simulink model "NBMS_SoC"  (R2026b)
settings: Solver=FixedStepDiscrete  StopTime=25  FixedStep=0.1
undefined symbols (not defined in the file): BMS_BattSoCDerate_E, BMS_BattTempDerate_E, BMS_MODE_E, CAL_15_SOC_WRN_RVL_THRSH, CAL_15_SOC_WRN_THRSH, CAL_DCHRG_END_THRSH, CAL_DOD, CAL_DOD_MAX_THRSH, CAL_DOD_MIN_THRSH, CAL_ENABLE_SOC_WARN_15, CAL_ENABLE_SOC_WARN_20, CAL_GOLDEN_CHARGE, CAL_GOLDEN_DC, CAL_LOW_SOC_RVL_THRSH, CAL_LOW_SOC_THRSH, CAL_NOMINAL_VOLTAGE, CAL_SOC_WRN_RVL_THRSH, CAL_SOC_WRN_THRSH, CAL_SOH_Enable, Charger_Mode_Req_E, DiscIntNeverNeededParam, OBC_E, VDU_MACHINE_STS_E, X_DCIR_CHG, X_DCIR_DISCH, Y_DCIR_CHG, Y_DCIR_DISCH
libraries: simulink x110, simulink_extras x6, sl_discontinuities x3
(part 2 of 3)

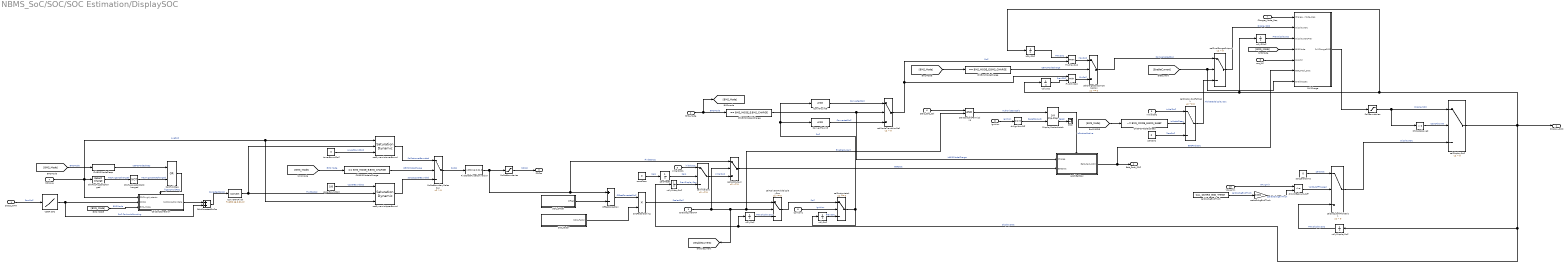
== system NBMS_SoC/SOC/SOC Estimation/DisplaySOC ==
  SOCcc_RAW : Inport
  BMS_Mode : Inport  Port=2
  EnableCurrentMA : Inport  Port=3
  SOCAvg : Inport  Port=4
  InitialSOC : Inport  Port=5
  Start_SOC_Cal : Inport  Port=6
  Charger_Mode_Req : Inport  Port=7
  Ignition : Inport  Port=8
  soc_full : Inport  Port=9
  VtAvgMin : Inport  Port=10
  CalcCorrectedSoCcc : Sum
  CalcSoCCorrection : Subsystem
  ChkBMSMODEIsSleep : simulink/Logic and Bit Operations/Compare To Constant  relop=~=  const=BMS_MODE_E.BMS_SLEEP  OutDataTypeStr=boolean
  ChkBMSModeIsCharge : simulink/Logic and Bit Operations/Compare To Constant  relop===  const=BMS_MODE_E.BMS_CHARGE  OutDataTypeStr=boolean
  ChkBMSModeSleep : simulink/Logic and Bit Operations/Compare To Constant  relop===  const=BMS_MODE_E.BMS_SLEEP  OutDataTypeStr=boolean
  ChkBMSModeisCharge : simulink/Logic and Bit Operations/Compare To Constant  relop===  const=BMS_MODE_E.BMS_CHARGE  OutDataTypeStr=boolean
  ChkBmsModeCharge : simulink/Logic and Bit Operations/Compare To Constant  relop===  const=BMS_MODE_E.BMS_CHARGE  OutDataTypeStr=boolean
  ChkHasAvgSoCChanged : simulink/Logic and Bit Operations/Detect Change  vinit=0  OutDataTypeStr=boolean
  ChkHasAvgSoCNotChanged : Logic  Operator=NOT  AllPortsSameDT=off  OutDataTypeStr=boolean
  ChkSoCabove0 : simulink/Logic and Bit Operations/Compare To Constant  relop=>  const=0  OutDataTypeStr=boolean
  ConvertToFixdt : DataTypeConversion  OutDataTypeStr=fixdt(0,16,0.01,0)  RndMeth=Floor
  ConvertTouin8 : DataTypeConversion  OutDataTypeStr=uint8  RndMeth=Ceiling
  ConvtTouint8 : DataTypeConversion  OutDataTypeStr=uint8  RndMeth=Floor
  DisplaySocLockLatch : simulink_extras/Flip Flops/S-R Flip-Flop  initial_condition=0
  FindMaxSoC : MinMax  Function=max  Inputs=2
  FindMinSoC : MinMax  Inputs=2
  FixdtDataTypeConversion : DataTypeConversion  OutDataTypeStr=fixdt(0,16,0.01,0)  RndMeth=Floor
  FullCharge : Subsystem
  GND : Terminator
  Ignition1 : InportShadow  Port=8
  InitialSOC1 : InportShadow  Port=5
  LatchBattSoc : Subsystem
  LowerBoundSoC : Constant  Value=0  OutDataTypeStr=fixdt(0,16,0.01,0)
  OffsetCorrection : Sum  Inputs=+-
  SOC_Offset : Subsystem
  SOC_factor : Subsystem
  SoCBoundaries : Saturate  UpperLimit=100  LowerLimit=0  OutDataTypeStr=uint8  RndMeth=Ceiling
  SoCFactorScaling : Product
  SoCHoldReq : Logic  Operator=OR  AllPortsSameDT=off  OutDataTypeStr=boolean
  SoCZeroClamp : Constant  Value=0  OutDataTypeStr=uint8
  SoCccBoundaries : Saturate  UpperLimit=100  LowerLimit=0  RndMeth=Nearest
  SoCccBoundarySelection : Switch  Criteria=u2 > Threshold  SaturateOnIntegerOverflow=off  InputSameDT=off
  StartSocCalcPermissive : Logic  AllPortsSameDT=off  OutDataTypeStr=boolean
  UDlySOC : UnitDelay  SampleTime=-1
  USER SOC : Lookup_n-D  NumberOfTableDimensions=1  BreakpointsForDimension1=[0,100]  Table=[0,100]  InternalRulePriority=Speed  RndMeth=Simplest
  UdlySoc : UnitDelay  SampleTime=-1
  UpperBoundSoC : Constant  Value=100  OutDataTypeStr=fixdt(0,16,0.01,0)
  ZeroReset : UnitDelay  InitialCondition=1  SampleTime=-1
  ZeroSoC : Constant  Value=0  OutDataTypeStr=uint8
  calDischgEndThrsh : Constant  Value=CAL_DCHRG_END_THRSH
  chkIgnitionOff : simulink/Logic and Bit Operations/Compare To Constant  relop===  const=0  OutDataTypeStr=boolean
  chkVoltBelowCutoff : RelationalOperator  Operator=<=  OutDataTypeStr=boolean  RndMeth=Simplest  InputSameDT=off
  constZero : Constant  Value=0  OutDataTypeStr=boolean
  satDynamicLowerBound : sl_discontinuities/Saturation Dynamic  OutMin=[]  OutMax=[]  OutDataTypeStr=Inherit: Same as second input  OutDataType=fixdt(1, 16)  OutScaling=2^-10  DoSatur=off
  satDynamicUpperBound : sl_discontinuities/Saturation Dynamic  OutMin=[]  OutMax=[]  OutDataTypeStr=Inherit: Same as second input  OutDataType=fixdt(1, 16)  OutScaling=2^-10  DoSatur=off
  scaleDchgEndThrsh : Gain  Gain=0.001
  selActiveOrHoldDisplaySoc : Switch  Criteria=u2 ~= 0  SaturateOnIntegerOverflow=off  InputSameDT=off
  selChargeSocCompensation : Switch  Criteria=u2 ~= 0  SaturateOnIntegerOverflow=off  InputSameDT=off
  selDisplaySoC : Switch  Criteria=u2 > Threshold  SaturateOnIntegerOverflow=off  InputSameDT=off
  selDisplaySocFallback : Switch  Criteria=u2 ~= 0  SaturateOnIntegerOverflow=off  InputSameDT=off
  selFinalGaugeOutput : Switch  Criteria=u2 > Threshold  SaturateOnIntegerOverflow=off  InputSameDT=off
  selInitialSoc : Switch  Criteria=u2 ~= 0  SaturateOnIntegerOverflow=off  InputSameDT=off
  selModeTransitionRef : Switch  Criteria=u2 > Threshold  SaturateOnIntegerOverflow=off  InputSameDT=off
  selSoCOutput : Switch  Criteria=u2 ~= 0  SaturateOnIntegerOverflow=off  InputSameDT=off
  selSocCutoffArbitration : Switch  Criteria=u2 > Threshold  SaturateOnIntegerOverflow=off  InputSameDT=off
  selSocIgnLatch : Switch  Criteria=u2 ~= 0  SaturateOnIntegerOverflow=off  InputSameDT=off
  uDlySoC : UnitDelay  InitialCondition=100  SampleTime=-1
  udlyDSoC : UnitDelay  InitialCondition=100  SampleTime=-1
  udlyDislaySoC : UnitDelay  SampleTime=-1
  udlyDisplaySoC : UnitDelay  SampleTime=-1
  udlySoC : UnitDelay  SampleTime=-1
  Display_SOC : Outport
  Batt_Pack_SOC : Outport  Port=2
  SOCcc : Outport  Port=3
  wires:
  [BMS_Mode] -> ChkBMSModeSleep/1  "BMSMode"
  ChkBMSModeSleep/1 -> SoCHoldReq/1  "IsBMSModeSleep"
  SoCHoldReq/1 -> CalcSoCCorrection/Enable  "flgSoCHoldReq"
  ChkHasAvgSoCNotChanged/1 -> SoCHoldReq/2  "HasAvgSoCNotChanged"
  [BMS_Mode] -> CalcSoCCorrection/3(BMS_Mode)  "BMSMode"
  soc_full/1 -> FullCharge/5(soc_full)
  udlySoC/1 -> selSocIgnLatch/3  "PrevSoC"
  selActiveOrHoldDisplaySoc/1 -> selSocIgnLatch/1  "SoC"
  Ignition1/1 -> selSocIgnLatch/2  "Ignition"
  [BMS_Mode] -> FullCharge/4(BMSMode)
  selDisplaySocFallback/1 -> selFinalGaugeOutput/3  "ArbitratedDisplaySoc"
  ZeroSoC/1 -> selDisplaySocFallback/3  "ZeroSoC"
  InitialSOC/1 -> selDisplaySocFallback/1  "initialSoC"
  ChkBMSMODEIsSleep/1 -> selDisplaySocFallback/2  "IsModeSleep"
  [BMS_Mode] -> ChkBMSMODEIsSleep/1
  uDlySoC/1 -> selActiveOrHoldDisplaySoc/3  "PrevDisplaySoc"
  BMS_Mode/1 -> ChkBMSModeisCharge/1, [BMS_Mode]  "BMSMode"
  LatchBattSoc/1(Batt_Pack_SOC) -> FullCharge/6(Batt_Pack_SOC), Batt_Pack_SOC/1  "BattPackSoC"
  Ignition/1 -> chkIgnitionOff/1  "Ignition"
  chkIgnitionOff/1 -> DisplaySocLockLatch/2  "ResetSocLock"
  udlyDSoC/1 -> FullCharge/3(DisplaySOCPrev)  "PrevDisplaySoc"
  Charger_Mode_Req/1 -> FullCharge/1(Charger_Mode_Req)
  FullCharge/1(FullChargeSOC) -> SoCBoundaries/1
  ConvertToFixdt/1 -> satDynamicLowerBound/2, satDynamicUpperBound/2  "FixdtSoCcc"
  UpperBoundSoC/1 -> satDynamicUpperBound/1  "UpperBoundSoc"
  satDynamicUpperBound/1 -> SoCccBoundarySelection/3  "SoCccUpperBounded"
  LowerBoundSoC/1 -> satDynamicLowerBound/3  "LowerBoundSoC"
  CalcCorrectedSoCcc/1 -> ConvertToFixdt/1  "CorrectedSoCcc"
  satDynamicLowerBound/1 -> SoCccBoundarySelection/1  "SoCccLowerBounded"
  ChkBMSModeIsCharge/1 -> SoCccBoundarySelection/2  "IsBMSModeCharge"
  [BMS_Mode] -> ChkBMSModeIsCharge/1  "BMS Mode"
  StartSocCalcPermissive/1 -> DisplaySocLockLatch/1  "AuthorizeSocCalc"
  Start_SOC_Cal/1 -> StartSocCalcPermissive/1
  DisplaySocLockLatch/2 -> GND/1  "Reset"
  DisplaySocLockLatch/1 -> LatchBattSoc/Enable  "IsSocLockActive"
  selSoCOutput/1 -> LatchBattSoc/2(BattSOC)  "BattSoC"
  constZero/1 -> ZeroReset/1  "Zero"
  ZeroReset/1 -> selInitialSoc/2  "Zero"
  InitialSOC1/1 -> selInitialSoc/1  "initialSoC"
  selInitialSoc/1 -> selSoCOutput/3  "InitialSoC"
  ChkBMSModeisCharge/1 -> LatchBattSoc/1(Charge), selModeTransitionRef/2  "IsBMSModeCharge"
  SoCccBoundaries/1 -> SOCcc/1  "SOCcc"
  [EnableCurrent] -> selFinalGaugeOutput/2, FullCharge/7(Enable2sec)
  USER SOC/1 -> CalcCorrectedSoCcc/2, CalcSoCCorrection/2(SOCcc)  "SoC CoulombCounting"
  selFinalGaugeOutput/1 -> FullCharge/2(DisplaySOC)  "DisplaySOC"
  selChargeSocCompensation/1 -> selFinalGaugeOutput/1  "CompensatedSoc"
  UdlySoc/1 -> FindMinSoC/2  "PrevSOC"
  UDlySOC/1 -> FindMaxSoC/1  "PrevSoC"
  selModeTransitionRef/1 -> FindMaxSoC/2, FindMinSoC/1  "SoC"
  FindMinSoC/1 -> selChargeSocCompensation/3  "MinSoC"
  FindMaxSoC/1 -> selChargeSocCompensation/1  "MaxSoC"
  [BMS_Mode] -> ChkBmsModeCharge/1
  ChkBmsModeCharge/1 -> selChargeSocCompensation/2  "IsBmsModeCharge"
  CalcSoCCorrection/1(SoCCorrectionRate) -> CalcCorrectedSoCcc/1
  ChkHasAvgSoCChanged/1 -> ChkHasAvgSoCNotChanged/1  "HasAvgSoCChanged"
  udlyDislaySoC/1 -> selInitialSoc/3  "PrevDisplaySoc"
  FixdtDataTypeConversion/1 -> OffsetCorrection/1, selSoCOutput/1, SoCccBoundaries/1  "FixdtSoCcc"
  ConvertTouin8/1 -> selModeTransitionRef/3  "ConvertedSoC"
  ConvtTouint8/1 -> selModeTransitionRef/1  "ConvertedSoC"
  selSocIgnLatch/1 -> ConvertTouin8/1, ConvtTouint8/1, udlySoC/1  "SoC"
  SoCFactorScaling/1 -> selActiveOrHoldDisplaySoc/1  "ScaledSoC"
  EnableCurrentMA/1 -> selSoCOutput/2, selActiveOrHoldDisplaySoc/2, StartSocCalcPermissive/2, [EnableCurrent]  "EnableCurrent"
  udlyDisplaySoC/1 -> selSocCutoffArbitration/3  "PrevDisplaySoC"
  SoCZeroClamp/1 -> selSocCutoffArbitration/1  "ZeroSoC"
  selSocCutoffArbitration/1 -> selDisplaySoC/3  "DisplaySOC"
  ChkSoCabove0/1 -> selDisplaySoC/2  "IsSoCAbove0"
  SoCBoundaries/1 -> ChkSoCabove0/1, selDisplaySoC/1  "DisplaySOC"
  SOCcc_RAW/1 -> USER SOC/1  "RawSoC"
  SOCAvg/1 -> ChkHasAvgSoCChanged/1, satDynamicLowerBound/1, satDynamicUpperBound/3, CalcSoCCorrection/1(SOCAvgHystersis)  "AvgSoC"
  selDisplaySoC/1 -> udlyDislaySoC/1, uDlySoC/1, udlyDisplaySoC/1, UDlySOC/1, udlyDSoC/1, UdlySoc/1, Display_SOC/1  "DisplaySOC"
  SOC_factor/1(SOC_Factor) -> SoCFactorScaling/2
  SOC_Offset/1(Offset) -> OffsetCorrection/2
  OffsetCorrection/1 -> SoCFactorScaling/1  "OffsetCorrectedSoC"
  SoCccBoundarySelection/1 -> FixdtDataTypeConversion/1  "SoCcc"
  calDischgEndThrsh/1 -> scaleDchgEndThrsh/1  "calDischgEndThrsh"
  scaleDchgEndThrsh/1 -> chkVoltBelowCutoff/2  "scaledDchgenThrsh"
  chkVoltBelowCutoff/1 -> selSocCutoffArbitration/2  "VoltCutoffTripped"
  VtAvgMin/1 -> chkVoltBelowCutoff/1  "VtAvgmin"

== system NBMS_SoC/SOC/SOC Estimation/LatchTempinit ==
  Temp : Inport
  Ignition : TriggerPort  VariantControl=(inherit)
  Temp_Init : Outport
  wires:
  Temp/1 -> Temp_Init/1

== system NBMS_SoC/SOC/SOC Estimation/SOC Overriding Handling ==
  soc_full : Inport
  Real_SOC : Inport  Port=2
  DisCharging_SOC : Inport  Port=3
  Charger_Mode_Req : Inport  Port=4
  BMS_Mode : Inport  Port=5
  CalcChgSoC : Sum  Inputs=+-
  ChkBMSModeSleep : simulink/Logic and Bit Operations/Compare To Constant  relop===  const=BMS_MODE_E.BMS_SLEEP  OutDataTypeStr=boolean
  ChkChgModeReqChgComplete : simulink/Logic and Bit Operations/Compare To Constant  relop===  const=Charger_Mode_Req_E.Charge_Complete  OutDataTypeStr=boolean
  ChkChgModeReqDisabled : simulink/Logic and Bit Operations/Compare To Constant  relop===  const=Charger_Mode_Req_E.Disabled  OutDataTypeStr=boolean
  LatchSoC : Subsystem  TreatAsAtomicUnit=on
  SoCccBoundaries : Saturate  UpperLimit=100  LowerLimit=0  OutDataTypeStr=double  RndMeth=Nearest
  SocStateController : Stateflow chart  TreatAsAtomicUnit=on
      settings: PortSchema="{\"entries\":[{\"content\":{\"sides\":[{\"content\":{\"connectorIds\":[\"In2\",\"In3\",\"In1\"]},\"type\":\"ConnectorPlacement.EquallySpacedRectSide\",\"uuid\":\"4d9dda48-5fd1-41f9-94f0-c80678ed5835\"},{\"content\":{\"connectorIds\":[\"Out1\"],\"side\":\"RIGHT\"},\"type\":\"ConnectorPlacement.EquallySpacedRectSide\",\"uuid\":\"c790fe46-1928-4eaf-b04a-be0eaec66a70\"},{\"content\":{\"side\":\"TOP\"},\"type\":\"ConnectorPlacement.EquallySpacedRectSide\",\"uuid\":\"e10142f7-42dd-412d-a45a-7f68ca23bebc\"},{\"content\":{\"side\":\"BOTTOM\"},\"type\":\"ConnectorPlacement.EquallySpacedRectSide\",\"uuid\":\"e986da1d-d2bc-437c-8de3-8b77989038a9\"}]},\"type\":\"ConnectorPlacement.EquallySpacedConnector\",\"uuid\":\"0a51b432-3f9b-4bde-863c-799f895a3b2c\"}],\"packageUris\":[\"http://schema.mathworks.com/mf0/Connector/R2020b\"],\"version\":\"1.0\"}"
  selChgOrRealSoc : Switch  Criteria=u2 > Threshold  SaturateOnIntegerOverflow=off  InputSameDT=off
  SOC_CC : Outport
  wires:
  CalcChgSoC/1 -> selChgOrRealSoc/1  "ChgSoC"
  LatchSoC/1(SOC) -> CalcChgSoC/1
  soc_full/1 -> LatchSoC/1(SOC_Full)  "SoCfull"
  ChkBMSModeSleep/1 -> SocStateController/3(BMS_sleep)  "IsBmsModeSleep"
  BMS_Mode/1 -> ChkBMSModeSleep/1
  SoCccBoundaries/1 -> SOC_CC/1  "SoCcc"
  selChgOrRealSoc/1 -> SoCccBoundaries/1  "UncappedSoCcc"
  Charger_Mode_Req/1 -> ChkChgModeReqChgComplete/1, ChkChgModeReqDisabled/1  "ChgModeReq"
  ChkChgModeReqDisabled/1 -> SocStateController/2(D)  "IsChgModeReqDisabled"
  SocStateController/1(A) -> selChgOrRealSoc/2  "SocSourceControl"
  Real_SOC/1 -> selChgOrRealSoc/3  "SoC"
  DisCharging_SOC/1 -> CalcChgSoC/2  "DischgSoc"
  ChkChgModeReqChgComplete/1 -> SocStateController/1(C), LatchSoC/Trigger  "IsChgModeReqChgComplete"

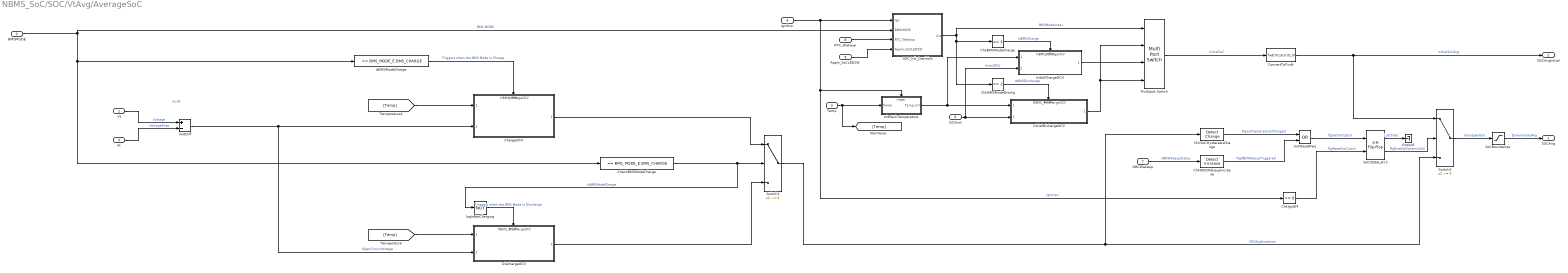
== system NBMS_SoC/SOC/VtAvg/AverageSoC ==
  note: Vt-IR
  Vt : Inport
  BMSMODE : Inport  Port=2
  Temp : Inport  Port=3  OutDataTypeStr=double
  Ignition : Inport  Port=4
  IR : Inport  Port=5
  OCVInit : Inport  Port=6
  OBCWakeup : Inport  Port=7
  RTC_Wakeup : Inport  Port=8
  AppIn_SoCLEDSW : Inport  Port=9
  ChargeOCV : ModelReference  ModelNameDialog=NBMS_ChargeOCV.slx  SimulationMode=Normal  ModelReferenceVersion=7.15  EnablePortName=EnableWhenValid  EnablePortStatesWhenEnabling=reset
  CheckBMSModeCharge : simulink/Logic and Bit Operations/Compare To Constant  relop===  const=BMS_MODE_E.BMS_CHARGE  OutDataTypeStr=boolean
  ChkBMSModeCharge : simulink/Logic and Bit Operations/Compare To Constant  relop===  const=1  OutDataTypeStr=boolean
  ChkBMSModeDischg : simulink/Logic and Bit Operations/Compare To Constant  relop===  const=2  OutDataTypeStr=boolean
  ChkIgnOff : simulink/Logic and Bit Operations/Compare To Zero  relop===  OutDataTypeStr=boolean
  ChkOBCWakeupIncrease : simulink/Logic and Bit Operations/Detect Increase  vinit=0.0  OutDataTypeStr=boolean
  ChkSoCHysteresisChange : simulink/Logic and Bit Operations/Detect Change  vinit=0  OutDataTypeStr=boolean
  ConvertToFixdt : DataTypeConversion  OutDataTypeStr=fixdt(0,16,0.01,0)  SaturateOnIntegerOverflow=off  RndMeth=Floor
  DischargeOCV : ModelReference  ModelNameDialog=NBMS_DischargeOCV.slx  SimulationMode=Normal  ModelReferenceVersion=7.7  EnablePortName=EnableWhenValid  EnablePortStatesWhenEnabling=reset
  Ground : Terminator
  InitPackTemperature : Subsystem  TreatAsAtomicUnit=on
  InitialChargeOCV : ModelReference  ModelNameDialog=NBMS_ChargeOCV.slx  SimulationMode=Normal  ModelReferenceVersion=7.15  EnablePortName=EnableWhenValid  EnablePortStatesWhenEnabling=reset
  InitialDichargeOCV : ModelReference  ModelNameDialog=NBMS_DischargeOCV.slx  SimulationMode=Normal  ModelReferenceVersion=7.7  EnablePortName=EnableWhenValid  EnablePortStatesWhenEnabling=reset
  IsBMSModeCharge : simulink/Logic and Bit Operations/Compare To Constant  relop===  const=BMS_MODE_E.BMS_CHARGE  OutDataTypeStr=boolean
  Multiport Switch : MultiPortSwitch  DataPortOrder=Zero-based contiguous  DiagnosticForDefault=None  zeroidx=on  SaturateOnIntegerOverflow=off  InputSameDT=off
  SOC_Init_Decision : Stateflow chart  TreatAsAtomicUnit=on
  SoCBoundaries : Saturate  UpperLimit=100  LowerLimit=0  RndMeth=Nearest
  SoCResetReq : Logic  Operator=OR  AllPortsSameDT=off  OutDataTypeStr=boolean
  SoCStateLatch : simulink_extras/Flip Flops/S-R Flip-Flop  initial_condition=0
  Switch1 : Switch  Criteria=u2 ~= 0  OutDataTypeStr=fixdt(0,16,0.01,0)  SaturateOnIntegerOverflow=off  InputSameDT=off
  Switch2 : Switch  Criteria=u2 ~= 0  SaturateOnIntegerOverflow=off  InputSameDT=off
  VoltDiff : Sum  Inputs=+-  OutDataTypeStr=fixdt(1,16,0.001,0)  AccumDataTypeStr=fixdt(1,16,0.001,0)
  logIsNotCharging : Logic  Operator=NOT  AllPortsSameDT=off  OutDataTypeStr=boolean
  SOCAvg : Outport
  SOCAvgInitial : Outport  Port=2
  wires:
  Vt/1 -> VoltDiff/1  "Voltage"
  OCVInit/1 -> InitialDichargeOCV/2, InitialChargeOCV/2  "InitialOCV"
  ChkIgnOff/1 -> SoCStateLatch/2  "flgResetSoCLatch"
  ChkBMSModeCharge/1 -> InitialChargeOCV/Enable  "IsBMSCharge"
  ChkOBCWakeupIncrease/1 -> SoCResetReq/2  "FlgOBCWakeupTriggered"
  SoCBoundaries/1 -> SOCAvg/1  "DynamicSoCAvg"
  ChkBMSModeDischg/1 -> InitialDichargeOCV/Enable  "IsBMSDischarge"
  SoCStateLatch/2 -> Switch2/2  "FlgEnableDynamicSoC"
  SoCStateLatch/1 -> Ground/1  "LatchSet"
  BMSMODE/1 -> CheckBMSModeCharge/1, IsBMSModeCharge/1, SOC_Init_Decision/2(BMSMODE)  "BMS MODE"
  Switch1/1 -> Switch2/3, ChkSoCHysteresisChange/1  "SOCAvgHystersis"
  Multiport Switch/1 -> ConvertToFixdt/1  "InitialSoC"
  SOC_Init_Decision/1(Init) -> Multiport Switch/1, ChkBMSModeCharge/1, ChkBMSModeDischg/1  "BMSModeIndex"
  ChkSoCHysteresisChange/1 -> SoCResetReq/1  "FlgSoCHysteresisIsChanged"
  ConvertToFixdt/1 -> Switch2/1, SOCAvgInitial/1  "InitialSoCAvg"
  [Temp] -> ChargeOCV/1
  VoltDiff/1 -> ChargeOCV/2, DischargeOCV/2  "OpenCircuitVoltage"
  Switch2/1 -> SoCBoundaries/1  "UncappedSoc"
  OBCWakeup/1 -> ChkOBCWakeupIncrease/1  "OBCWakeupStatus"
  IR/1 -> VoltDiff/2  "VoltageDrop"
  Ignition/1 -> InitPackTemperature/Trigger, ChkIgnOff/1, SOC_Init_Decision/1(Ign)  "Ignition"
  CheckBMSModeCharge/1 -> logIsNotCharging/1, Switch1/2  "IsBMSModeCharge"
  [Temp] -> DischargeOCV/1
  logIsNotCharging/1 -> DischargeOCV/Enable  "Triggers when the BMS Mode is Discharge"
  IsBMSModeCharge/1 -> ChargeOCV/Enable  "Triggers when the BMS Mode is Charge"
  Temp/1 -> InitPackTemperature/1(Temp), [Temp]
  SoCResetReq/1 -> SoCStateLatch/1  "flgSetSoCLatch"
  InitPackTemperature/1(Temp_Init) -> InitialDichargeOCV/1, InitialChargeOCV/1
  ChargeOCV/1 -> Switch1/1
  DischargeOCV/1 -> Switch1/3
  InitialChargeOCV/1 -> Multiport Switch/3
  InitialDichargeOCV/1 -> Multiport Switch/2, Multiport Switch/4
  RTC_Wakeup/1 -> SOC_Init_Decision/3(RTC_Wakeup)
  AppIn_SoCLEDSW/1 -> SOC_Init_Decision/4(AppIn_SoCLEDSW)

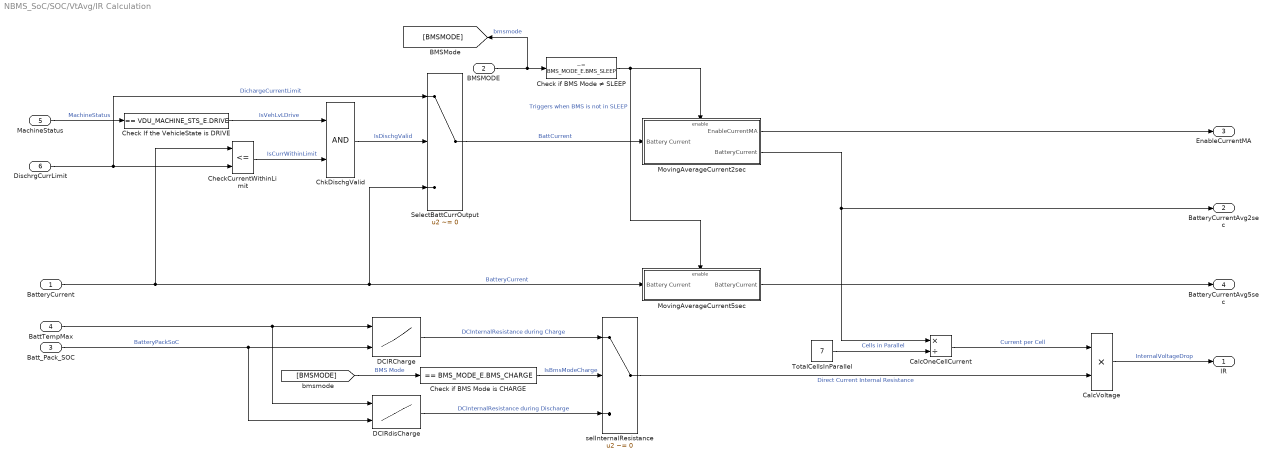
== system NBMS_SoC/SOC/VtAvg/IR Calculation ==
  BatteryCurrent : Inport
  BMSMODE : Inport  Port=2
  Batt_Pack_SOC : Inport  Port=3
  BattTempMax : Inport  Port=4
  MachineStatus : Inport  Port=5  OutDataTypeStr=Enum: VDU_MACHINE_STS_E
  DischrgCurrLimit : Inport  Port=6
  CalcOneCellCurrent : Product  Inputs=*/
  CalcVoltage : Product
  Check If the VehicleState is DRIVE : simulink/Logic and Bit Operations/Compare To Constant  relop===  const=VDU_MACHINE_STS_E.DRIVE  OutDataTypeStr=boolean
  "Check if BMS Mode ≠ SLEEP " : simulink/Logic and Bit Operations/Compare To Constant  relop=~=  const=BMS_MODE_E.BMS_SLEEP  OutDataTypeStr=boolean
  Check if BMS Mode is CHARGE : simulink/Logic and Bit Operations/Compare To Constant  relop===  const=BMS_MODE_E.BMS_CHARGE  OutDataTypeStr=boolean
  CheckCurrentWithinLimit : RelationalOperator  Operator=<=  OutDataTypeStr=boolean  RndMeth=Simplest  InputSameDT=off
  ChkDischgValid : Logic  AllPortsSameDT=off  OutDataTypeStr=boolean
  DCIRCharge : Lookup_n-D  BreakpointsForDimension1=X_DCIR_CHG  BreakpointsForDimension2=Y_DCIR_CHG  Table=[0.1796 0.1796 0.1427 0.2163 0.2033 0.2013 0.2128 0.2128 0.2128 0.2128 0.2128;0.0883 0.0883 0.0672 0.1006 0.0948 0.0949 0.1067 0.1035 0.1035 0.1035 0.1035;0.0742 0.0742 0.0579 0.0531 0.0482 0.0485 0.0584 0.0576 0.0631 0.0631 0.0631;0.0554 0.0554 0.0407 0.0412 0.038 0.039 0.0386 0.0389 0.0429 0.0402 0.0402;0.059 0.0414 0.0282 0.0291 0.0272 0.0277 0.0285 0.0271 0.0286 0.0269 0.0269;0.0479 0.0358 0.0221 0.0233 0.0215 0.0217 0.0218 0.0212 0.022 0.0195 0.0195;0.0448 0.0327 0.02 0.0219 0.0202 0.0204 0.0205 0.0195 0.0206 0.0181 0.0181]  ExtrapMethod=Clip  InternalRulePriority=Speed  OutDataTypeStr=Inherit: Inherit via back propagation  RndMeth=Simplest  InputSameDT=off
      settings: InputPortMap=u0,u1
  DCIRdisCharge : Lookup_n-D  BreakpointsForDimension1=X_DCIR_DISCH  BreakpointsForDimension2=Y_DCIR_DISCH  Table=[0.4429 0.4429 0.1677 0.1473 0.1409 0.1403 0.1384 0.1409 0.1428 0.1421 0.151;0.2169 0.2169 0.0906 0.0755 0.0721 0.0709 0.0713 0.0732 0.0738 0.0709 0.0772;0.1281 0.1281 0.0657 0.0554 0.053 0.053 0.0526 0.0531 0.0556 0.0525 0.0558;0.0808 0.0808 0.0453 0.0396 0.0389 0.0387 0.0385 0.0396 0.0407 0.038 0.0417;0.1135 0.0531 0.0333 0.029 0.0284 0.0284 0.028 0.0284 0.0299 0.0277 0.0296;0.0885 0.0407 0.0269 0.0233 0.0227 0.0229 0.0219 0.0228 0.0239 0.021 0.0234;0.086 0.0373 0.025 0.0221 0.022 0.0218 0.0207 0.0214 0.0224 0.0195 0.022]  ExtrapMethod=Clip  InternalRulePriority=Speed  OutDataTypeStr=Inherit: Inherit via back propagation  RndMeth=Simplest  InputSameDT=off
      settings: InputPortMap=u0,u1
  MovingAverageCurrent2sec : Subsystem
  MovingAverageCurrent5sec : Subsystem
  SelectBattCurrOutput : Switch  Criteria=u2 ~= 0  SaturateOnIntegerOverflow=off  InputSameDT=off
  TotalCellsInParallel : Constant  Value=7
  selInternalResistance : Switch  Criteria=u2 ~= 0  SaturateOnIntegerOverflow=off  InputSameDT=off
  IR : Outport
  BatteryCurrentAvg2sec : Outport  Port=2  OutDataTypeStr=fixdt(1,16,0.01,0)
  EnableCurrentMA : Outport  Port=3  OutDataTypeStr=boolean
  BatteryCurrentAvg5sec : Outport  Port=4  OutDataTypeStr=fixdt(1,16,0.01,0)
  wires:
  BattTempMax/1 -> DCIRCharge/1, DCIRdisCharge/1
  CheckCurrentWithinLimit/1 -> ChkDischgValid/2  "IsCurrWithinLimit"
  "Check if BMS Mode ≠ SLEEP "/1 -> MovingAverageCurrent5sec/Enable, MovingAverageCurrent2sec/Enable  "Triggers when BMS is not in SLEEP"
  DischrgCurrLimit/1 -> SelectBattCurrOutput/1, CheckCurrentWithinLimit/2  "DichargeCurrentLimit"
  CalcOneCellCurrent/1 -> CalcVoltage/1  "Current per Cell"
  selInternalResistance/1 -> CalcVoltage/2  "Direct Current Internal Resistance"
  CalcVoltage/1 -> IR/1  "InternalVoltageDrop"
  MovingAverageCurrent5sec/1(BatteryCurrent) -> BatteryCurrentAvg5sec/1
  DCIRCharge/1 -> selInternalResistance/1  "DCInternalResistance during Charge"
  DCIRdisCharge/1 -> selInternalResistance/3  "DCInternalResistance during Discharge"
  Batt_Pack_SOC/1 -> DCIRCharge/2, DCIRdisCharge/2  "BatteryPackSoC"
  [BMSMODE] -> Check if BMS Mode is CHARGE/1  "BMS Mode"
  TotalCellsInParallel/1 -> CalcOneCellCurrent/2  "Cells in Parallel"
  ChkDischgValid/1 -> SelectBattCurrOutput/2  "IsDischgValid"
  SelectBattCurrOutput/1 -> MovingAverageCurrent2sec/1(Battery Current)  "BattCurrent"
  Check If the VehicleState is DRIVE/1 -> ChkDischgValid/1  "IsVehLvLDrive"
  BatteryCurrent/1 -> SelectBattCurrOutput/3, MovingAverageCurrent5sec/1(Battery Current), CheckCurrentWithinLimit/1  "BatteryCurrent"
  Check if BMS Mode is CHARGE/1 -> selInternalResistance/2  "IsBmsModeCharge"
  BMSMODE/1 -> "Check if BMS Mode ≠ SLEEP "/1, [BMSMODE]  "bmsmode"
  MovingAverageCurrent2sec/2(BatteryCurrent) -> CalcOneCellCurrent/1, BatteryCurrentAvg2sec/1
  MachineStatus/1 -> Check If the VehicleState is DRIVE/1  "MachineStatus"
  MovingAverageCurrent2sec/1(EnableCurrentMA) -> EnableCurrentMA/1

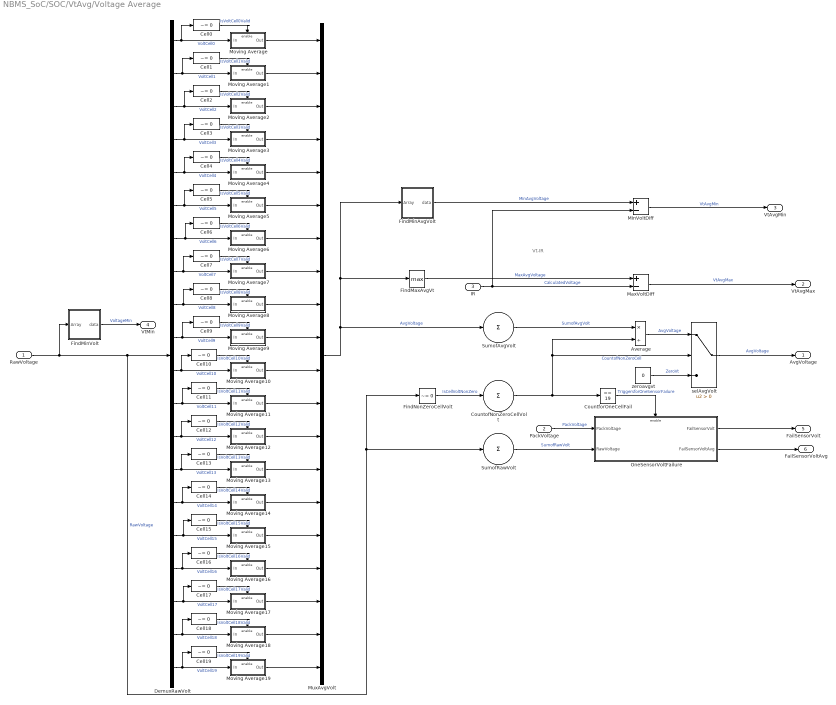
== system NBMS_SoC/SOC/VtAvg/Voltage Average ==
  note: Vt-IR
  RawVoltage : Inport
  PackVoltage : Inport  Port=2
  IR : Inport  Port=3
  Average : Product  Inputs=*/  OutDataTypeStr=fixdt(0,16,0.01,0)
  Cell{0..19} (20 alike) : simulink/Logic and Bit Operations/Compare To Zero  relop=~=  OutDataTypeStr=boolean
  CountforOneCellFail : simulink/Logic and Bit Operations/Compare To Constant  relop===  const=19  OutDataTypeStr=boolean
  CountofNonZeroCellVolt : Sum  Inputs=+  OutDataTypeStr=double  SaturateOnIntegerOverflow=on
  DemuxRawVolt : Demux  Outputs=20
  FindMaxAvgVt : MinMax  Function=max
  FindMinAvgVolt : Stateflow chart  TreatAsAtomicUnit=on
  FindMinVolt : Stateflow chart  TreatAsAtomicUnit=on
  FindNonZeroCellVolt : simulink/Logic and Bit Operations/Compare To Constant  relop=~=  const=0  OutDataTypeStr=boolean
  MaxVoltDiff : Sum  Inputs=+-  OutDataTypeStr=fixdt(1,16,0.001,0)  AccumDataTypeStr=fixdt(1,16,0.001,0)
  MinVoltDiff : Sum  Inputs=+-  OutDataTypeStr=fixdt(1,16,0.001,0)  AccumDataTypeStr=fixdt(1,16,0.001,0)
  Moving Average : Subsystem
  Moving Average1 : Subsystem
  Moving Average10 : Subsystem
  Moving Average11 : Subsystem
  Moving Average12 : Subsystem
  Moving Average13 : Subsystem
  Moving Average14 : Subsystem
  Moving Average15 : Subsystem
  Moving Average16 : Subsystem
  Moving Average17 : Subsystem
  Moving Average18 : Subsystem
  Moving Average19 : Subsystem
  Moving Average2 : Subsystem
  Moving Average3 : Subsystem
  Moving Average4 : Subsystem
  Moving Average5 : Subsystem
  Moving Average6 : Subsystem
  Moving Average7 : Subsystem
  Moving Average8 : Subsystem
  Moving Average9 : Subsystem
  MuxAvgVolt : Mux  Inputs=20
  OneSensorVoltFailure : Subsystem  TreatAsAtomicUnit=on
  SumofAvgVolt : Sum  Inputs=+  OutDataTypeStr=double  SaturateOnIntegerOverflow=on
  SumofRawVolt : Sum  Inputs=+  OutDataTypeStr=double  SaturateOnIntegerOverflow=on
  selAvgVolt : Switch  Criteria=u2 > Threshold  SaturateOnIntegerOverflow=off  InputSameDT=off
  zeroavgvt : Constant  Value=0
  AvgVoltage : Outport
  VtAvgMax : Outport  Port=2
  VtAvgMin : Outport  Port=3
  VtMin : Outport  Port=4
  FailSensorVolt : Outport  Port=5  OutputWhenDisabled=reset  InitialOutput=5
  FailSensorVoltAvg : Outport  Port=6  OutputWhenDisabled=reset  InitialOutput=5
  wires:
  SumofAvgVolt/1 -> Average/1  "SumofAvgVolt"
  DemuxRawVolt/1 -> Cell0/1, Moving Average/1(In)  "VoltCell0"
  FindMinVolt/1(data) -> VtMin/1  "VoltageMin"
  OneSensorVoltFailure/1(FailSensorVolt) -> FailSensorVolt/1
  DemuxRawVolt/12 -> Moving Average11/1(In), Cell11/1  "VoltCell11"
  SumofRawVolt/1 -> OneSensorVoltFailure/2(RawVoltage)  "SumofRawVolt"
  DemuxRawVolt/17 -> Moving Average16/1(In), Cell16/1  "VoltCell16"
  Cell12/1 -> Moving Average12/Enable  "IsVoltCell12Valid"
  Moving Average6/1(Out) -> MuxAvgVolt/7
  Moving Average19/1(Out) -> MuxAvgVolt/20
  DemuxRawVolt/3 -> Moving Average2/1(In), Cell2/1  "VoltCell2"
  DemuxRawVolt/11 -> Moving Average10/1(In), Cell10/1  "VoltCell10"
  Moving Average5/1(Out) -> MuxAvgVolt/6
  OneSensorVoltFailure/2(FailSensorVoltAvg) -> FailSensorVoltAvg/1
  Cell10/1 -> Moving Average10/Enable  "IsVoltCell10Valid"
  DemuxRawVolt/13 -> Moving Average12/1(In), Cell12/1  "VoltCell12"
  Cell14/1 -> Moving Average14/Enable  "IsVoltCell14Valid"
  Cell9/1 -> Moving Average9/Enable  "IsVoltCell9Valid"
  Cell16/1 -> Moving Average16/Enable  "IsVoltCell16Valid"
  Cell15/1 -> Moving Average15/Enable  "IsVoltCell15Valid"
  DemuxRawVolt/20 -> Moving Average19/1(In), Cell19/1  "VoltCell19"
  Moving Average15/1(Out) -> MuxAvgVolt/16
  DemuxRawVolt/14 -> Moving Average13/1(In), Cell13/1  "VoltCell13"
  MaxVoltDiff/1 -> VtAvgMax/1  "VtAvgMax"
  DemuxRawVolt/16 -> Moving Average15/1(In), Cell15/1  "VoltCell15"
  Cell2/1 -> Moving Average2/Enable  "IsVoltCell2Valid"
  FindMinAvgVolt/1(data) -> MinVoltDiff/1  "MinAvgVoltage"
  Cell13/1 -> Moving Average13/Enable  "IsVoltCell13Valid"
  DemuxRawVolt/2 -> Moving Average1/1(In), Cell1/1  "VoltCell1"
  Cell1/1 -> Moving Average1/Enable  "IsVoltCell1Valid"
  DemuxRawVolt/5 -> Moving Average4/1(In), Cell4/1  "VoltCell4"
  Moving Average17/1(Out) -> MuxAvgVolt/18
  Cell7/1 -> Moving Average7/Enable  "IsVoltCell7Valid"
  Cell8/1 -> Moving Average8/Enable  "IsVoltCell8Valid"
  DemuxRawVolt/15 -> Moving Average14/1(In), Cell14/1  "VoltCell14"
  MuxAvgVolt/1 -> FindMinAvgVolt/1(Array), FindMaxAvgVt/1, SumofAvgVolt/1  "AvgVoltage"
  CountforOneCellFail/1 -> OneSensorVoltFailure/Enable  "TriggersforOneSensorFailure"
  RawVoltage/1 -> FindMinVolt/1(Array), FindNonZeroCellVolt/1, SumofRawVolt/1, DemuxRawVolt/1  "RawVoltage"
  MinVoltDiff/1 -> VtAvgMin/1  "VtAvgMin"
  IR/1 -> MinVoltDiff/2, MaxVoltDiff/2  "CalculatedVoltage"
  CountofNonZeroCellVolt/1 -> Average/2, selAvgVolt/2, CountforOneCellFail/1  "CountofNonZeroCell"
  Cell6/1 -> Moving Average6/Enable  "IsVoltCell6Valid"
  DemuxRawVolt/6 -> Moving Average5/1(In), Cell5/1  "VoltCell5"
  Moving Average3/1(Out) -> MuxAvgVolt/4
  FindMaxAvgVt/1 -> MaxVoltDiff/1  "MaxAvgVoltage"
  PackVoltage/1 -> OneSensorVoltFailure/1(PackVoltage)  "PackVoltage"
  Cell11/1 -> Moving Average11/Enable  "IsVoltCell11Valid"
  DemuxRawVolt/19 -> Moving Average18/1(In), Cell18/1  "VoltCell18"
  DemuxRawVolt/18 -> Moving Average17/1(In), Cell17/1  "VoltCell17"
  DemuxRawVolt/8 -> Moving Average7/1(In), Cell7/1  "VoltCell7"
  Cell18/1 -> Moving Average18/Enable  "IsVoltCell18Valid"
  Moving Average11/1(Out) -> MuxAvgVolt/12
  DemuxRawVolt/10 -> Moving Average9/1(In), Cell9/1  "VoltCell9"
  Moving Average14/1(Out) -> MuxAvgVolt/15
  Moving Average1/1(Out) -> MuxAvgVolt/2
  Moving Average7/1(Out) -> MuxAvgVolt/8
  Moving Average13/1(Out) -> MuxAvgVolt/14
  DemuxRawVolt/7 -> Moving Average6/1(In), Cell6/1  "VoltCell6"
  Moving Average18/1(Out) -> MuxAvgVolt/19
  Moving Average/1(Out) -> MuxAvgVolt/1
  FindNonZeroCellVolt/1 -> CountofNonZeroCellVolt/1  "IsCellVoltNonZero"
  Cell4/1 -> Moving Average4/Enable  "IsVoltCell4Valid"
  Cell5/1 -> Moving Average5/Enable  "IsVoltCell5Valid"
  DemuxRawVolt/4 -> Moving Average3/1(In), Cell3/1  "VoltCell3"
  Moving Average16/1(Out) -> MuxAvgVolt/17
  Cell3/1 -> Moving Average3/Enable  "IsVoltCell3Valid"
  DemuxRawVolt/9 -> Moving Average8/1(In), Cell8/1  "VoltCell8"
  Cell0/1 -> Moving Average/Enable  "IsVoltCell0Valid"
  Cell17/1 -> Moving Average17/Enable  "IsVoltCell17Valid"
  Moving Average12/1(Out) -> MuxAvgVolt/13
  Cell19/1 -> Moving Average19/Enable  "IsVoltCell19Valid"
  Moving Average8/1(Out) -> MuxAvgVolt/9
  Moving Average2/1(Out) -> MuxAvgVolt/3
  Moving Average9/1(Out) -> MuxAvgVolt/10
  Moving Average10/1(Out) -> MuxAvgVolt/11
  Moving Average4/1(Out) -> MuxAvgVolt/5
  Average/1 -> selAvgVolt/1  "AvgVoltage"
  selAvgVolt/1 -> AvgVoltage/1  "AvgVoltage"
  zeroavgvt/1 -> selAvgVolt/3  "ZeroVt"

== system NBMS_SoC/SOC/LifeCycle SOH Energy/State of Health/CalcChgMeasured ==
  BatteryCurrent : Inport
  ChrgMeasureTrig : Inport  Port=2
  Enable : EnablePort
  Absolute : Abs  SaturateOnIntegerOverflow=off
  CalcAccumulatedBattCurr : DiscreteIntegrator  ExternalReset=rising  SampleTime=-1  ICPrevOutput=DiscIntNeverNeededParam  ICPrevScaledInput=DiscIntNeverNeededParam
  scaleBattCurr : Gain  Gain=1000
  secPerHour : Gain  Gain=1/3600
  Output : Outport
  wires:
  CalcAccumulatedBattCurr/1 -> scaleBattCurr/1  "AccumulatedBatteryCurrent"
  ChrgMeasureTrig/1 -> CalcAccumulatedBattCurr/2  "IsChargeMeasureTriggered"
  BatteryCurrent/1 -> Absolute/1  "BattCurr"
  Absolute/1 -> secPerHour/1  "AbsBattCurr"
  secPerHour/1 -> CalcAccumulatedBattCurr/1  "BattCurrAh"
  scaleBattCurr/1 -> Output/1  "ChargeMeasured"

== system NBMS_SoC/SOC/LifeCycle SOH Energy/State of Health/CalculateSoH ==
  Charg_measured : Inport
  Charg_capacity : Inport  Port=2
  SoC_Start : Inport  Port=3
  CalcDOD : Sum  Inputs=+-
  CalcDischgCapacity : Product
  CalcMinSoH : MinMax  Inputs=2
  CalcSoH : Product  Inputs=*/
  MaxSoC : Constant  Value=100
  MaxSoH : Constant  Value=100
  scaleMeasuredCharge : Gain  Gain=100*100
  SoH : Outport
  wires:
  Charg_measured/1 -> scaleMeasuredCharge/1  "MeasuredCharge"
  SoC_Start/1 -> CalcDOD/2  "SoCatStart"
  MaxSoC/1 -> CalcDOD/1  "MaxSoC"
  CalcDOD/1 -> CalcDischgCapacity/2  "DODatStart"
  Charg_capacity/1 -> CalcDischgCapacity/1  "ChargeCapacity"
  scaleMeasuredCharge/1 -> CalcSoH/1  "ScaledCharge"
  CalcDischgCapacity/1 -> CalcSoH/2  "Capacity"
  CalcSoH/1 -> CalcMinSoH/1  "New_SoH"
  MaxSoH/1 -> CalcMinSoH/2  "MaxSoH"
  CalcMinSoH/1 -> SoH/1  "SoH"

== system NBMS_SoC/SOC/LifeCycle SOH Energy/State of Health/Initial_SoC_Storage ==
  Display_SOC : Inport
  TriggerWhenChargeHasinitiated : TriggerPort  VariantControl=(inherit)
  SoC_Start : Outport
  wires:
  Display_SOC/1 -> SoC_Start/1  "SoCStart"

== system NBMS_SoC/SOC/SOC Estimation/CurrentCapacityCalculation/LatchInitCapacity ==
  CurrCapacity : Inport
  Trigger : TriggerPort  VariantControl=(inherit)
  LatchedCapacity : Outport
  wires:
  CurrCapacity/1 -> LatchedCapacity/1  "InitialCapacity"

== system NBMS_SoC/SOC/SOC Estimation/DisplaySOC/CalcSoCCorrection ==
  SOCAvgHystersis : Inport
  SOCcc : Inport  Port=2
  BMS_Mode : Inport  Port=3
  EnableBlock : EnablePort
  ChkBMSModeIsSleep : simulink/Logic and Bit Operations/Compare To Constant  relop===  const=BMS_MODE_E.BMS_SLEEP  OutDataTypeStr=boolean
  ClampZero : Constant  Value=0
  HoldZero : Constant  Value=0
  ScaleSoCError : Product  Inputs=*/
  SecperHour : Constant  Value=36000
  SoCAccumulate : Sum
  SoCDeviation : Sum  Inputs=+-
  SocCorrectionLimits : sl_discontinuities/Saturation Dynamic  OutMin=[]  OutMax=[]  OutDataTypeStr=Inherit: Same as second input  OutDataType=fixdt(1, 16)  OutScaling=2^-10  DoSatur=off
  ZeroHold : Constant  Value=0
  selLowerBoundaryCheck : Switch  SaturateOnIntegerOverflow=off  InputSameDT=off
  selSleepStateFallBack : Switch  Criteria=u2 ~= 0  SaturateOnIntegerOverflow=off  InputSameDT=off
  selUpperBoundaryCheck : Switch  SaturateOnIntegerOverflow=off  InputSameDT=off
  udlySoCError : UnitDelay  SampleTime=-1
  SoCCorrectionRate : Outport  InitialOutput=0
  wires:
  udlySoCError/1 -> selSleepStateFallBack/3  "PrevSoCError"
  ZeroHold/1 -> selSleepStateFallBack/1
  selSleepStateFallBack/1 -> SoCAccumulate/2  "ArbitratedSoC"
  ChkBMSModeIsSleep/1 -> selSleepStateFallBack/2  "IsBMSModeSleep"
  BMS_Mode/1 -> ChkBMSModeIsSleep/1  "BMSMode"
  SOCcc/1 -> SoCDeviation/2  "SoCCoulombCount"
  SecperHour/1 -> ScaleSoCError/2  "secperHour"
  SOCAvgHystersis/1 -> SoCDeviation/1  "SoCAvgHysteresis"
  ScaleSoCError/1 -> SoCAccumulate/1  "ScaledSoCError"
  SocCorrectionLimits/1 -> SoCCorrectionRate/1  "SoCCorrection"
  SoCAccumulate/1 -> SocCorrectionLimits/2, udlySoCError/1  "SoCAccumulateError"
  SoCDeviation/1 -> selLowerBoundaryCheck/2, selLowerBoundaryCheck/3, selUpperBoundaryCheck/2, selUpperBoundaryCheck/1, ScaleSoCError/1  "SoCError"
  selUpperBoundaryCheck/1 -> SocCorrectionLimits/1  "UpperBoundCorrection"
  selLowerBoundaryCheck/1 -> SocCorrectionLimits/3  "LowerBoundCorrection"
  ClampZero/1 -> selUpperBoundaryCheck/3  "ClampZeroRef"
  HoldZero/1 -> selLowerBoundaryCheck/1  "HoldZeroRef"

== system NBMS_SoC/SOC/SOC Estimation/DisplaySOC/FullCharge ==
  Charger_Mode_Req : Inport
  DisplaySOC : Inport  Port=2
  DisplaySOCPrev : Inport  Port=3
  BMSMode : Inport  Port=4
  soc_full : Inport  Port=5
  Batt_Pack_SOC : Inport  Port=6
  Enable2sec : Inport  Port=7
  ChargeCompletionTrigger : Logic  AllPortsSameDT=off  OutDataTypeStr=boolean
  ChgTerminationLt : Constant  Value=99  OutDataTypeStr=Inherit: Inherit via back propagation
  ChkChgModeReqChgComplete : simulink/Logic and Bit Operations/Compare To Constant  relop===  const=Charger_Mode_Req_E.Charge_Complete  OutDataTypeStr=boolean
  Detect Increase : simulink/Logic and Bit Operations/Detect Increase  vinit=0.0  OutDataTypeStr=boolean
  LatchFullSoc : Subsystem  TreatAsAtomicUnit=on
  MaxSOC : Constant  Value=100  OutDataTypeStr=Inherit: Inherit via back propagation
  MaxSoC : Constant  Value=100  OutDataTypeStr=Inherit: Inherit via back propagation
  PackTopOffCondition : Logic  Inputs=3  AllPortsSameDT=off  OutDataTypeStr=boolean
  StateWaitCondition : Stateflow chart  TreatAsAtomicUnit=on
  chkDisplaySocAtMax : RelationalOperator  Operator===  OutDataTypeStr=boolean  RndMeth=Simplest  InputSameDT=off
  chkIsModeCharge : simulink/Logic and Bit Operations/Compare To Constant  relop===  const=BMS_MODE_E.BMS_CHARGE  OutDataTypeStr=boolean
  chkPackSocBelowFull : simulink/Logic and Bit Operations/Compare To Constant  relop=<=  const=99  OutDataTypeStr=boolean
  chkPrevStateComplete : RelationalOperator  Operator===  OutDataTypeStr=boolean  RndMeth=Simplest  InputSameDT=off
  selDisplaySocFallback : Switch  Criteria=u2 ~= 0  SaturateOnIntegerOverflow=off  InputSameDT=off
  selFullChargeSocSource : Switch  Criteria=u2 ~= 0  SaturateOnIntegerOverflow=off  InputSameDT=off
  selTerminationSocRef : Switch  Criteria=u2 ~= 0  SaturateOnIntegerOverflow=off  InputSameDT=off
  udlyEnableCurrent : UnitDelay  SampleTime=-1
  FullChargeSOC : Outport
  wires:
  selTerminationSocRef/1 -> selFullChargeSocSource/3  "TerminationSocRef"
  MaxSOC/1 -> chkDisplaySocAtMax/2  "SoCMax"
  ChkChgModeReqChgComplete/1 -> Detect Increase/1  "IsChgModeReqChgComplete"
  soc_full/1 -> LatchFullSoc/1(SOC_Full)  "SoCFull"
  LatchFullSoc/1(SOC) -> selFullChargeSocSource/1
  ChargeCompletionTrigger/1 -> selDisplaySocFallback/2  "ChargeCompletePulse"
  chkIsModeCharge/1 -> ChargeCompletionTrigger/2  "IsBMSModeCharge"
  chkDisplaySocAtMax/1 -> ChargeCompletionTrigger/1  "IsSoCatMax"
  BMSMode/1 -> chkIsModeCharge/1  "BmsMode"
  selFullChargeSocSource/1 -> FullChargeSOC/1  "FullChargeSoC"
  DisplaySOC/1 -> chkPrevStateComplete/1, selDisplaySocFallback/3, chkDisplaySocAtMax/1
  Charger_Mode_Req/1 -> ChkChgModeReqChgComplete/1  "ChargerModeReq"
  chkPackSocBelowFull/1 -> PackTopOffCondition/1  "IsPackSoCBelowFull"
  chkPrevStateComplete/1 -> PackTopOffCondition/2  "IsPrevStateComplete"
  PackTopOffCondition/1 -> selTerminationSocRef/2  "PackTopOffDetected"
  Batt_Pack_SOC/1 -> chkPackSocBelowFull/1  "BattPackSOC"
  ChgTerminationLt/1 -> selTerminationSocRef/1  "ChrgTerminationLimit"
  DisplaySOCPrev/1 -> selDisplaySocFallback/1  "PrevDisplaySoC"
  MaxSoC/1 -> chkPrevStateComplete/2  "SoCMax"
  selDisplaySocFallback/1 -> selTerminationSocRef/3  "ArbitratedDisplaySoc"
  Enable2sec/1 -> StateWaitCondition/1(Enable), udlyEnableCurrent/1  "EnableCurrent"
  StateWaitCondition/1(out) -> PackTopOffCondition/3  "HoldState"
  udlyEnableCurrent/1 -> StateWaitCondition/2(prev)  "PrevEnable"
  Detect Increase/1 -> LatchFullSoc/Trigger, selFullChargeSocSource/2

== system NBMS_SoC/SOC/SOC Estimation/DisplaySOC/LatchBattSoc ==
  Charge : Inport
  BattSOC : Inport  Port=2
  Enable : EnablePort
  BattSoCBoundaries : Saturate  UpperLimit=100  LowerLimit=0  OutDataTypeStr=double  RndMeth=Ceiling
  FindMax : MinMax  Function=max  Inputs=2
  FindMin : MinMax  Inputs=2
  selBattSoC : Switch  Criteria=u2 > Threshold  SaturateOnIntegerOverflow=off  InputSameDT=off
  uDlyBattSoC : UnitDelay  SampleTime=-1
  udlyBattSoC : UnitDelay  InitialCondition=100  SampleTime=-1
  Batt_Pack_SOC : Outport  InitialOutput=0
  wires:
  BattSoCBoundaries/1 -> Batt_Pack_SOC/1  "Batt_Pack_SOC"
  BattSOC/1 -> FindMin/1, FindMax/2  "BattSoC"
  FindMax/1 -> selBattSoC/1  "SoCMaxValue"
  FindMin/1 -> selBattSoC/3  "SoCMinValue"
  Charge/1 -> selBattSoC/2
  uDlyBattSoC/1 -> FindMax/1  "PrevBattSoC"
  udlyBattSoC/1 -> FindMin/2  "PrevBattSoC"
  selBattSoC/1 -> udlyBattSoC/1, BattSoCBoundaries/1, uDlyBattSoC/1  "UncappedBattSoC"

== system NBMS_SoC/SOC/SOC Estimation/DisplaySOC/SOC_Offset ==
  CalDODMinThrsh : Constant  Value=CAL_DOD_MIN_THRSH
  CalcOffset : Product  Inputs=*/
  DODThrshDiff : Sum  Inputs=+-
  ScaleMinThrsh : Product
  ScalingFactor : Constant  Value=100
  calDODMaxThrsh : Constant  Value=CAL_DOD_MAX_THRSH
  calDODMinThrsh : Constant  Value=CAL_DOD_MIN_THRSH
  Offset : Outport
  wires:
  ScalingFactor/1 -> ScaleMinThrsh/1  "ScaleFactor"
  CalcOffset/1 -> Offset/1  "CalculatedOffset"
  CalDODMinThrsh/1 -> ScaleMinThrsh/2  "DODMinThrsh"
  ScaleMinThrsh/1 -> CalcOffset/1  "ScaledMinThrsh"
  calDODMinThrsh/1 -> DODThrshDiff/2  "DODMinThrsh"
  DODThrshDiff/1 -> CalcOffset/2  "DODThrshDelta"
  calDODMaxThrsh/1 -> DODThrshDiff/1  "DODMaxThrsh"

== system NBMS_SoC/SOC/SOC Estimation/DisplaySOC/SOC_factor ==
  CalcSoCFactor : Product  Inputs=*/
  DODThrshDiff : Sum  Inputs=+-
  ScalingFactor : Constant  Value=100
  calDODMaxThrsh : Constant  Value=CAL_DOD_MAX_THRSH
  calDODMinThrsh : Constant  Value=CAL_DOD_MIN_THRSH
  SOC_Factor : Outport
  wires:
  calDODMinThrsh/1 -> DODThrshDiff/2  "DODMinThrsh"
  DODThrshDiff/1 -> CalcSoCFactor/2  "DODThrshDiff"
  calDODMaxThrsh/1 -> DODThrshDiff/1  "DODMaxThrsh"
  CalcSoCFactor/1 -> SOC_Factor/1  "SoCFactor"
  ScalingFactor/1 -> CalcSoCFactor/1  "ScaledFactor"

== system NBMS_SoC/SOC/SOC Estimation/SOC Overriding Handling/LatchSoC ==
  SOC_Full : Inport
  Trigger : TriggerPort  VariantControl=(inherit)  PortDimensions=1
  SOC : Outport  InitialOutput=0
  wires:
  SOC_Full/1 -> SOC/1  "SoC"

== system NBMS_SoC/SOC/VtAvg/AverageSoC/InitPackTemperature ==
  Temp : Inport
  TrigWhenValid : TriggerPort  VariantControl=(inherit)
  Temp_Init : Outport
  wires:
  Temp/1 -> Temp_Init/1  "Initial Temp"

== system NBMS_SoC/SOC/VtAvg/IR Calculation/MovingAverageCurrent2sec ==
  note: 2 sec holding the average
  Battery Current : Inport
  Enable : EnablePort  StatesWhenEnabling=reset
  1UnitDelay : UnitDelay  SampleTime=-1
  20Delay : simulink/Discrete/Tapped Delay  vinit=0.0  samptime=0.1  NumDelays=20  DelayOrder=Oldest  includeCurrent=off
  Average : Product  Inputs=*/  OutDataTypeStr=fixdt(1,16,0.01,0)
  "CheckBufferComplete  " : simulink/Logic and Bit Operations/Compare To Constant  relop=>  const=20  OutDataTypeStr=boolean
  ConstZeroCurrent : Constant  Value=0  OutDataTypeStr=fixdt(1,16,0.01,0)
  ConvertToFixdt : DataTypeConversion  OutDataTypeStr=fixdt(1,16,0.01,0)  SaturateOnIntegerOverflow=off  RndMeth=Floor
  CountStep : Constant  OutDataTypeStr=uint8
  Counter : Sum  AccumDataTypeStr=uint8  SaturateOnIntegerOverflow=on
  "Sample Accumulator " : Switch  Criteria=u2 ~= 0  Threshold=20  SaturateOnIntegerOverflow=off  InputSameDT=off
  Sumof21Samples : Sum  OutDataTypeStr=fixdt(1,32,0.01,0)  AccumDataTypeStr=fixdt(1,32,0.01,0)
  SumofCurrent : Sum  Inputs=+  OutDataTypeStr=fixdt(1,32,0.01,0)  AccumDataTypeStr=fixdt(1,32,0.01,0)
  TotalCount : Constant  Value=21  OutDataTypeStr=fixdt(1,16,0.01,0)
  EnableCurrentMA : Outport  OutDataTypeStr=boolean  OutputWhenDisabled=reset  InitialOutput=0
  BatteryCurrent : Outport  Port=2  OutputWhenDisabled=reset  InitialOutput=0
  wires:
  "CheckBufferComplete  "/1 -> EnableCurrentMA/1, "Sample Accumulator "/2  "EnableCurrent"
  ConstZeroCurrent/1 -> "Sample Accumulator "/3  "ZeroCurrent"
  Counter/1 -> 1UnitDelay/1, "CheckBufferComplete  "/1  "CounterValue"
  TotalCount/1 -> Average/2  "TotalSampleCount"
  SumofCurrent/1 -> Sumof21Samples/1  "AccumulatedSumof20Samples"
  20Delay/1 -> SumofCurrent/1  "CurrentSampleDelayed20"
  Sumof21Samples/1 -> Average/1  "SumofallCurrent"
  Battery Current/1 -> ConvertToFixdt/1  "BatteryCurrent"
  CountStep/1 -> Counter/1  "CounterIncrement"
  "Sample Accumulator "/1 -> BatteryCurrent/1  "2secAvgBatteryCurrent"
  1UnitDelay/1 -> Counter/2  "PreviousValue"
  ConvertToFixdt/1 -> 20Delay/1, Sumof21Samples/2  "21stSample"
  Average/1 -> "Sample Accumulator "/1  "AverageCurrent"

== system NBMS_SoC/SOC/VtAvg/IR Calculation/MovingAverageCurrent5sec ==
  note: 5 sec holding the average
  Battery Current : Inport
  EnableBlock : EnablePort  StatesWhenEnabling=reset
  1UnitDelay : UnitDelay  SampleTime=-1
  50Delay : simulink/Discrete/Tapped Delay  vinit=0.0  samptime=0.1  NumDelays=50  DelayOrder=Oldest  includeCurrent=off
  Average : Product  Inputs=*/  OutDataTypeStr=fixdt(1,16,0.01,0)
  CheckBufferComplete : simulink/Logic and Bit Operations/Compare To Constant  relop=>  const=50  OutDataTypeStr=boolean
  ConstZeroCurrent : Constant  Value=0  OutDataTypeStr=fixdt(1,16,0.01,0)
  ConvertToFixdt : DataTypeConversion  OutDataTypeStr=fixdt(1,16,0.01,0)  SaturateOnIntegerOverflow=off  RndMeth=Floor
  CountStep : Constant  OutDataTypeStr=uint8
  Counter : Sum  AccumDataTypeStr=uint8  SaturateOnIntegerOverflow=on
  "Sample Accumulator " : Switch  Criteria=u2 ~= 0  Threshold=20  SaturateOnIntegerOverflow=off  InputSameDT=off
  Sumof51Samples : Sum  OutDataTypeStr=fixdt(1,32,0.01,0)  AccumDataTypeStr=fixdt(1,32,0.01,0)
  SumofCurrent : Sum  Inputs=+  OutDataTypeStr=fixdt(1,32,0.01,0)  AccumDataTypeStr=fixdt(1,32,0.01,0)
  TotalCount : Constant  Value=51  OutDataTypeStr=fixdt(1,16,0.01,0)
  BatteryCurrent : Outport  OutputWhenDisabled=reset  InitialOutput=0
  wires:
  Average/1 -> "Sample Accumulator "/1  "CalcAverageCurrent"
  ConvertToFixdt/1 -> Sumof51Samples/2, 50Delay/1  "51stSample"
  1UnitDelay/1 -> Counter/2  "PreviousValue"
  "Sample Accumulator "/1 -> BatteryCurrent/1  "5secAvgBatteryCurrent"
  CountStep/1 -> Counter/1  "CounterIncrement"
  Battery Current/1 -> ConvertToFixdt/1  "BatteryCurrent"
  Sumof51Samples/1 -> Average/1  "SumofallCurrent"
  50Delay/1 -> SumofCurrent/1  "CurrentSampleDelayed50"
  SumofCurrent/1 -> Sumof51Samples/1  "AccumulatedSumof50Samples"
  TotalCount/1 -> Average/2  "TotalSampleCount"
  Counter/1 -> 1UnitDelay/1, CheckBufferComplete/1  "CountValue"
  ConstZeroCurrent/1 -> "Sample Accumulator "/3  "ZeroCurrent"
  CheckBufferComplete/1 -> "Sample Accumulator "/2  "IsSampleWindowFull"

== system NBMS_SoC/SOC/VtAvg/Voltage Average/Moving Average ==
  note: 2sec Holding the Average
  In : Inport
  EnableCellVoltValid : EnablePort
  20Delay : simulink/Discrete/Tapped Delay  vinit=0.0  samptime=-1  NumDelays=20  DelayOrder=Newest  includeCurrent=off
  Average : Product  Inputs=*/  OutDataTypeStr=fixdt(1,16,0.001,0)
  CountStep : Constant  OutDataTypeStr=uint8
  Counter : Sum  AccumDataTypeStr=uint8  SaturateOnIntegerOverflow=on
  Counterfor20 : Switch  Criteria=u2 > Threshold  Threshold=20  SaturateOnIntegerOverflow=off  InputSameDT=off
  Delayfor1Unit : UnitDelay  SampleTime=-1
  FixdtDataTypeConversion : DataTypeConversion  OutDataTypeStr=fixdt(1,16,0.001,0)  SaturateOnIntegerOverflow=off  RndMeth=Floor
  SumofVoltage : Sum  Inputs=+  OutDataTypeStr=fixdt(1,32,0.001,0)  AccumDataTypeStr=fixdt(1,32,0.001,0)
  TotalCount : Constant  Value=21  OutDataTypeStr=fixdt(1,16,0.001,0)
  TotalSum : Sum  OutDataTypeStr=fixdt(1,32,0.001,0)  AccumDataTypeStr=fixdt(1,32,0.001,0)
  ZeroVt : Constant  Value=0  OutDataTypeStr=fixdt(1,16,0.001,0)
  Out : Outport
  wires:
  Counter/1 -> Counterfor20/2, Delayfor1Unit/1  "CounterValue"
  FixdtDataTypeConversion/1 -> TotalSum/2, 20Delay/1  "21stVoltage"
  Counterfor20/1 -> Out/1  "AvgVoltofCell0"
  TotalSum/1 -> Average/1  "SumofallVolt"
  CountStep/1 -> Counter/1  "CounterIncrement"
  ZeroVt/1 -> Counterfor20/3  "ZeroVoltage"
  TotalCount/1 -> Average/2  "TotalSample"
  Delayfor1Unit/1 -> Counter/2  "PreviousValue"
  SumofVoltage/1 -> TotalSum/1  "AccumulatedSumof20Vt"
  In/1 -> FixdtDataTypeConversion/1  "VoltCell0"
  20Delay/1 -> SumofVoltage/1  "SampleDelayed20"
  Average/1 -> Counterfor20/1  "AverageVolt"

== system NBMS_SoC/SOC/VtAvg/Voltage Average/Moving Average1 ==
  note: 2sec Holding the Average
  In : Inport
  EnableCellVoltValid : EnablePort
  20Delay : simulink/Discrete/Tapped Delay  vinit=0.0  samptime=-1  NumDelays=20  DelayOrder=Newest  includeCurrent=off
  Average : Product  Inputs=*/  OutDataTypeStr=fixdt(1,16,0.001,0)
  CountStep : Constant  OutDataTypeStr=uint8
  Counter : Sum  AccumDataTypeStr=uint8  SaturateOnIntegerOverflow=on
  Counterfor20 : Switch  Criteria=u2 > Threshold  Threshold=20  SaturateOnIntegerOverflow=off  InputSameDT=off
  Delayfor1Unit : UnitDelay  SampleTime=-1
  FixdtDataTypeConversion : DataTypeConversion  OutDataTypeStr=fixdt(1,16,0.001,0)  SaturateOnIntegerOverflow=off  RndMeth=Floor
  SumofVoltage : Sum  Inputs=+  OutDataTypeStr=fixdt(1,32,0.001,0)  AccumDataTypeStr=fixdt(1,32,0.001,0)
  TotalCount : Constant  Value=21  OutDataTypeStr=fixdt(1,16,0.001,0)
  TotalSum : Sum  OutDataTypeStr=fixdt(1,32,0.001,0)  AccumDataTypeStr=fixdt(1,32,0.001,0)
  ZeroVt : Constant  Value=0  OutDataTypeStr=fixdt(1,16,0.001,0)
  Out : Outport
  wires:
  Average/1 -> Counterfor20/1  "AverageVolt"
  TotalCount/1 -> Average/2  "TotalSample"
  ZeroVt/1 -> Counterfor20/3  "ZeroVoltage"
  20Delay/1 -> SumofVoltage/1  "SampleDelayed20"
  Counter/1 -> Counterfor20/2, Delayfor1Unit/1  "CounterValue"
  In/1 -> FixdtDataTypeConversion/1  "VoltCell1"
  CountStep/1 -> Counter/1  "CounterIncrement"
  Delayfor1Unit/1 -> Counter/2  "PreviousValue"
  SumofVoltage/1 -> TotalSum/1  "AccumulatedSumof20Vt"
  TotalSum/1 -> Average/1  "SumofallVolt"
  Counterfor20/1 -> Out/1  "AvgVoltofCell1"
  FixdtDataTypeConversion/1 -> TotalSum/2, 20Delay/1  "21stVoltage"
